simulink model "CombGyroAccel_Filter"  (R2013b)
settings: Solver=FixedStepDiscrete  SolverMode=SingleTasking  StartTime=0.0  StopTime=inf  FixedStep=sim_step_size  RelTol=1e-3
PreLoadFcn:
  | Gyro_Bias = -247;
  | sim_step_size = 0.03;
undefined symbols (not defined in the file or in its folder): DiscIntNeverNeededParam
settings Model: SimulationMode=external  ExtModeTrigDuration=2  Creator=nding  LastModifiedBy=nding
settings OptimizationCC: OptimizeModelRefInitCode=on  LifeSpan=1
settings DebuggingCC: SolverPrmCheckMsg=none
settings HardwareCC: ProdBitPerInt=16  ProdBitPerPointer=8  ProdIntDivRoundTo=Zero  ProdEndianess=LittleEndian  ProdWordSize=8  ProdHWDeviceType=Atmel->AVR
settings RTWCC: SystemTargetFile=realtime.tlc  GenerateMakefile=off  TemplateMakefile=realtime.tmf  Description=Run on Target Hardware  RTWVerbose=off  ProcessScript=realtime_make_rtw_hook
settings STFCustomTargetCC: TargetLibSuffix=.a  GenerateSampleERTMain=on  ERTCustomFileBanners=on  SupportNonInlinedSFcns=off  SupportVariableSizeSignals=on  MATLABClassNameForMDSCustomization=Simulink.SoftwareTarget.ERTCustomization  GRTInterface=off  SystemTargetFile=realtime.tlc
settings ERTTargetCC: CodeReplacementLibrary=ANSI_C  GenerateSampleERTMain=on  ParMdlRefBuildCompliant=off  CompOptLevelCompliant=off  ConcurrentExecutionCompliant=off  CombineOutputUpdateFcns=off  ERTFirstTimeCompliant=off  SupportContinuousTime=on  SupportVariableSizeSignals=on  ModelStepFunctionPrototypeControlCompliant=off  CPPClassGenCompliant=off  ExtModeTransport=3  ExtModeMexFile=ext_serial_win32_comm  ExtModeMexArgs=0 1 9600  InlinedParameterPlacement=NonHierarchical  ERTSrcFileBannerTemplate=realtime_code_template.cgt  ERTHdrFileBannerTemplate=realtime_code_template.cgt  ERTDataSrcFileTemplate=realtime_code_template.cgt  ERTDataHdrFileTemplate=realtime_code_template.cgt  ERTCustomFileTemplate=realtime_file_process.tlc

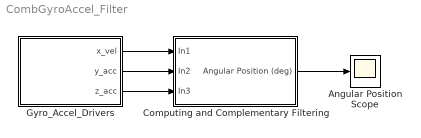
== system CombGyroAccel_Filter ==
  Angular Position Scope : Scope
      settings: TimeRange=25  YMin=-50  YMax=90
  Computing and Complementary Filtering : Subsystem
  Gyro_Accel_Drivers : Subsystem
  wires:
  Gyro_Accel_Drivers/1(x_vel) -> Computing and Complementary Filtering/1(In1)
  Gyro_Accel_Drivers/2(y_acc) -> Computing and Complementary Filtering/2(In2)
  Gyro_Accel_Drivers/3(z_acc) -> Computing and Complementary Filtering/3(In3)
  Computing and Complementary Filtering/1(Angular Position (deg)) -> Angular Position Scope/1

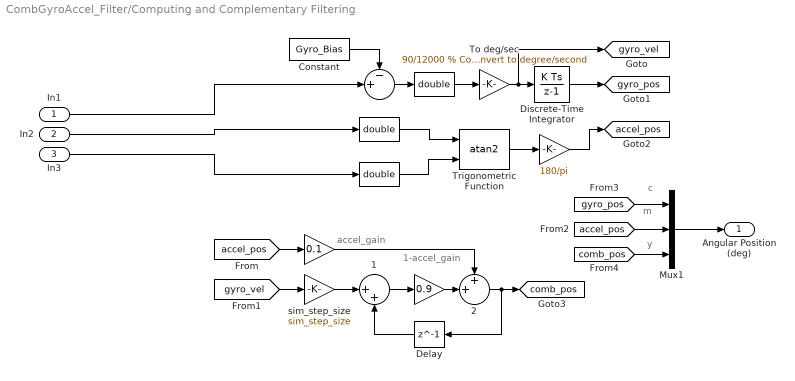
== system CombGyroAccel_Filter/Computing and Complementary Filtering ==
  note: 1-accel_gain
  note: accel_gain
  note: c
  note: m
  note: y
  In1 : Inport
  In2 : Inport  Port=2
  In3 : Inport  Port=3
  " " : Sum  Inputs=-+|
  "  " : DataTypeConversion  OutDataTypeStr=double
  "   " : DataTypeConversion  OutDataTypeStr=double
  "    " : Gain  Gain=0.1
  "     " : DataTypeConversion  OutDataTypeStr=double
  "      " : Gain  Gain=180/pi
  "          " : Gain  Gain=0.9
  "    sim_step_size" : Gain  Gain=sim_step_size
  " 1" : Sum  Inputs=|++
  " 2" : Sum  Inputs=++|
  Constant : Constant  Value=Gyro_Bias
  Delay : Delay  DelayLength=1
  Discrete-Time Integrator : DiscreteIntegrator  SampleTime=-1  ICPrevOutput=DiscIntNeverNeededParam  ICPrevScaledInput=DiscIntNeverNeededParam
  Mux1 : Mux  Inputs=3
  To deg/sec : Gain  Gain=90/12000 % Convert to degree/second
  Trigonometric Function : Trigonometry  Operator=atan2
  Angular Position (deg) : Outport
  tag scope: accel_pos=global, comb_pos=global, gyro_pos=global, gyro_vel=global
  wires:
  In2/1 -> "   "/1
  In3/1 -> "     "/1
  In1/1 -> " "/2
  Trigonometric Function/1 -> "      "/1
  [comb_pos] -> Mux1/3
  [gyro_vel] -> "    sim_step_size"/1
  "   "/1 -> Trigonometric Function/1
  Discrete-Time Integrator/1 -> [gyro_pos]
  [accel_pos] -> Mux1/2
  "      "/1 -> [accel_pos]
  "     "/1 -> Trigonometric Function/2
  Mux1/1 -> Angular Position (deg)/1
  "  "/1 -> To deg/sec/1
  "    "/1 -> " 2"/1
  Constant/1 -> " "/1
  "          "/1 -> " 2"/2
  To deg/sec/1 -> Discrete-Time Integrator/1, [gyro_vel]
  [gyro_pos] -> Mux1/1
  " 2"/1 -> Delay/1, [comb_pos]
  "    sim_step_size"/1 -> " 1"/1
  Delay/1 -> " 1"/2
  " "/1 -> "  "/1
  " 1"/1 -> "          "/1
  [accel_pos] -> "    "/1

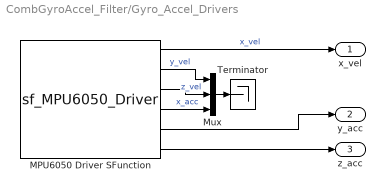
== system CombGyroAccel_Filter/Gyro_Accel_Drivers ==
  MPU6050 Driver SFunction : S-Function  InitFcn=try, set_param(gcb,'FunctionName','sf_MPU6050_Driver'), end  FunctionName=sf_MPU6050_Driver  SFunctionModules=sf_MPU6050_Driver_wrapper  EnableBusSupport=off  mask(S-Function Builder){}
      mask help: Simulink:masks:SFunctionBuilder_MD
      mask init:
      | val = [[.9  0.75 0.75 1 1 .9 .9 1]',[1 1 0.75 0.75 .9 .9 1 .9]'];try , sys = get_param(gcb,'SfunBuilderFcnName');if isempty(sys), sys = get_param(gcb,'FunctionName'); end,catch, sys = get_param(gcb,'FunctionName'); end
      settings: CopyFcn=set_param(gcbh,'LinkStatus','none')  PreSaveFcn=try, set_param(gcb,'FunctionName','sf_MPU6050_Driver'), end  OpenFcn=sfunctionwizard(gcbh)
      mask Display: plot(val(:,1),val(:,2)),disp(sys), port_label('output',1,'x_vel'), port_label('output',2,'y_vel'), port_label('output',3,'z_vel'), port_label('output',4,'x_acc'), port_label('output',5,'y_acc'), port_label('output',6,'z_acc')
  Mux : Mux  Inputs=3
  Terminator : Terminator
  x_vel : Outport
  y_acc : Outport  Port=2
  z_acc : Outport  Port=3
  wires:
  Mux/1 -> Terminator/1
  MPU6050 Driver SFunction/4 -> Mux/3  "x_acc"
  MPU6050 Driver SFunction/5 -> y_acc/1
  MPU6050 Driver SFunction/6 -> z_acc/1
  MPU6050 Driver SFunction/1 -> x_vel/1  "x_vel"
  MPU6050 Driver SFunction/2 -> Mux/1  "y_vel"
  MPU6050 Driver SFunction/3 -> Mux/2  "z_vel"
